simulink model "robotLQG_sim"  (R2026b)
settings: Solver=ode45  StopTime=Tstop  MaxStep=0.002  RelTol=1e-6
PreLoadFcn:
  | robotLQG_setup_AIgen;
InitFcn:
  | robotLQG_setup_AIgen;
values from neighbouring files (symbols this model uses):
  alphaMax = lim.alphaMax    [robotLQG_setup_AIgen.m]    (also in stepperLimits_AIgen.m = alphaBox(k))
  gyroNoiseVar = sensorNonIdeal*sigGyro^2    (= 1.21846967915e-05)    [robotLQG_setup_AIgen.m]
  K = lqrd(Ai, Bi, Q, R, Ts)    [robotLQG_setup_AIgen.m]    (also in robotPoleExplorer_AIgen.m = lqr(me.A, me.B, Q, Rw); solveDARE_AIgen.m = (R + B'*P*B) \ (B'*P*A + N'))
  kest = kalmd(ss(A1,[B1, B1],C1,zeros(2,2)),1/24,((pi/180)^2)*[1/24 0; 0 5E-6],Ts)    [controller_lqg_ia.m]    (also in discreteKalman_AIgen.m = struct('A', Ad - L*C, 'B', [Bd - L*D, L], 'L', L,           ; robotLQG_setup_AIgen.m = kalmd(ss(A, [B, G], C, [D, zeros(3, 2)]), Qn, Rn, Ts))
  omegaMax = lim.omegaMax    [robotLQG_setup_AIgen.m]    (also in stepperLimits_AIgen.m = w(k))
  p = struct('mc', mc, 'Jc', Jc, 'mw', mw, 'Jw', Jw, 'l', l, 'r', r,                         'g', 9.81,                         'Jr', 2*Jrotor,                         'b_phi', 0,                         'b_theta', 0)    [classBalancingRobotFlowLinear_AIgen.m]    (also in classBalancingRobotRigLinear_AIgen.m = classBalancingRobotFlowLinear_AIgen.estimatedParameters(); fitRigFall_AIgen.m = c(nRun + 1:end); robotLQG_setup_AIgen.m = [robot.mc; robot.Jc; robot.mw; robot.Jw; robot.l; robot.r; r)
  phiRefRate = 2    [robotLQG_setup_AIgen.m]
  phiRefStepTime = 3    [robotLQG_setup_AIgen.m]
  thetaBiasUsed = sensorNonIdeal*thetaBias    (= 0.0261799387799)    [robotLQG_setup_AIgen.m]
  thetaNoiseVar = sensorNonIdeal*sigTheta^2    (= 1.21846967915e-05)    [robotLQG_setup_AIgen.m]
  Ts = 0.002    [robotLQG_setup_AIgen.m]
  x0 = [0; theta0; obj.momentum(0, dtheta0)]    [classBalancingRobotRigLinear_AIgen.m]    (also in robotLQG_setup_AIgen.m = [0; 5*pi/180; 0])
  xhat0 = [0; x0(2) + thetaBiasUsed; 0]    [robotLQG_setup_AIgen.m]
  zLimit = 0.5*alphaMax/abs(Kz)    [robotLQG_setup_AIgen.m]
undefined symbols (not defined in the file or in its folder): DiscIntNeverNeededParam
settings Model: Creator=61404  LastModifiedBy=61404

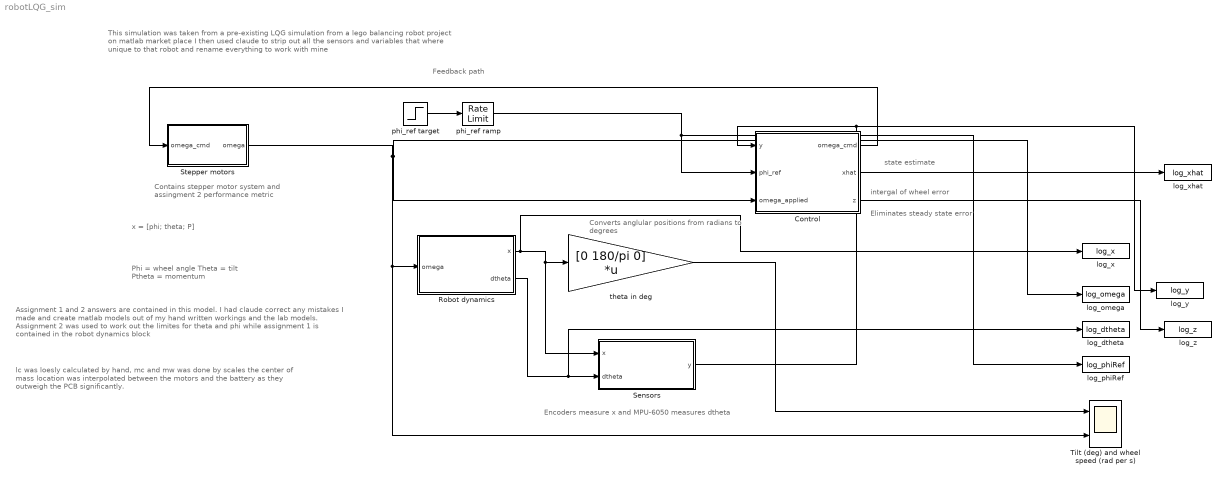
== system robotLQG_sim ==
  note: lc was loesly calculated by hand, mc and mw was done by scales
      | the center of mass location was interpolated between the motors and the
      | battery as they outweigh the PCB significantly.
  note: Assignment 1 and 2 answers are contained in this model.
      | I had claude correct any mistakes I made and create matlab models out of my
      | hand written workings and the lab models. Assignment 2 was used to work out
      | the limites for theta and phi while assignment 1 is contained in the robot dynamics block
  note: Eliminates steady state error
  note: intergal of wheel error
  note: state estimate
  note: Phi = wheel angle
      | Theta = tilt
      | Ptheta = momentum
  note: x = [phi;
      | 	theta;
      | 	P]
  note: This simulation was taken from a pre-existing LQG simulation from a lego balancing robot project on matlab market place
      | I then used claude to strip out all the sensors and variables that where unique to that robot and rename everything to work with mine
  note: Encoders measure x and MPU-6050 measures dtheta
  note: Feedback path
  note: Converts anglular positions from radians to
      | degrees
  note: Contains stepper motor system
      | and assingment 2 performance metric
  Control : Subsystem
  Robot dynamics : Subsystem
  Sensors : Subsystem
  Stepper motors : Subsystem
  Tilt (deg) and wheel speed (rad per s) : Scope  NumInputPorts=2
  log_dtheta : ToWorkspace  VariableName=log_dtheta  SaveFormat=Structure With Time  SampleTime=Ts
  log_omega : ToWorkspace  VariableName=log_omega  SaveFormat=Structure With Time  SampleTime=Ts
  log_phiRef : ToWorkspace  VariableName=log_phiRef  SaveFormat=Structure With Time  SampleTime=Ts
  log_x : ToWorkspace  VariableName=log_x  SaveFormat=Structure With Time  SampleTime=Ts
  log_xhat : ToWorkspace  VariableName=log_xhat  SaveFormat=Structure With Time  SampleTime=Ts
  log_y : ToWorkspace  VariableName=log_y  SaveFormat=Structure With Time  SampleTime=Ts
  log_z : ToWorkspace  VariableName=log_z  SaveFormat=Structure With Time  SampleTime=Ts
  phi_ref ramp : RateLimiter  RisingSlewLimit=phiRefRate  FallingSlewLimit=-phiRefRate  SampleTimeMode=inherited
  phi_ref target : Step  Time=phiRefStepTime  FinalValue=phiRefStep  SampleTime=Ts
  theta in deg : Gain  Gain=[0 180/pi 0]  Multiplication=Matrix(K*u)
  wires:
  Robot dynamics/1(x) -> Sensors/1(x), theta in deg/1, log_x/1
  Stepper motors/1(omega) -> Tilt (deg) and wheel speed (rad per s)/2, Robot dynamics/1(omega), Control/3(omega_applied), log_omega/1
  phi_ref target/1 -> phi_ref ramp/1
  Sensors/1(y) -> Control/1(y), log_y/1
  Control/1(omega_cmd) -> Stepper motors/1(omega_cmd)
  Robot dynamics/2(dtheta) -> Sensors/2(dtheta), log_dtheta/1
  phi_ref ramp/1 -> Control/2(phi_ref), log_phiRef/1
  theta in deg/1 -> Tilt (deg) and wheel speed (rad per s)/1
  Control/2(xhat) -> log_xhat/1
  Control/3(z) -> log_z/1

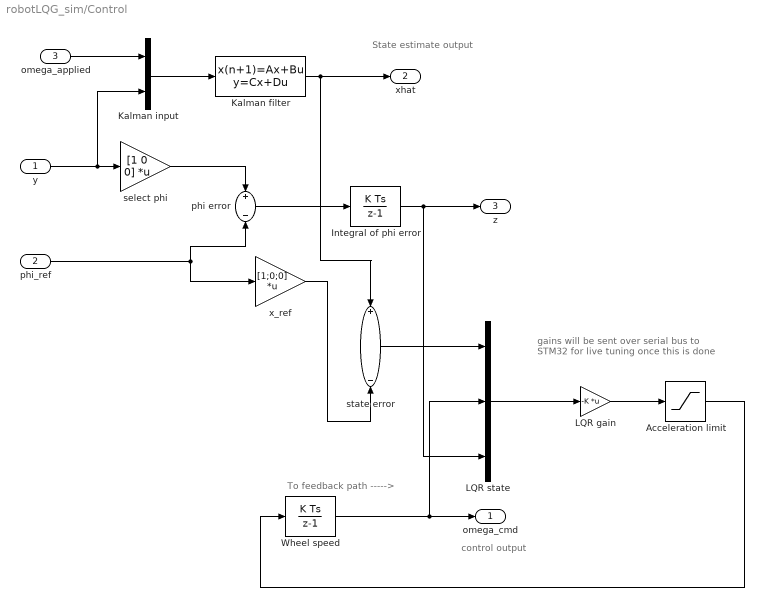
== system robotLQG_sim/Control ==
  note: State estimate output
  note: control output
  note: To feedback path ----->
  note: gains will be sent over serial bus to
      | STM32 for live tuning once this is done
  y : Inport
  phi_ref : Inport  Port=2
  omega_applied : Inport  Port=3
  Acceleration limit : Saturate  UpperLimit=alphaMax  LowerLimit=-alphaMax
  Integral of phi error : DiscreteIntegrator  SampleTime=Ts  LimitOutput=on  UpperSaturationLimit=zLimit  LowerSaturationLimit=-zLimit  ICPrevOutput=DiscIntNeverNeededParam  ICPrevScaledInput=DiscIntNeverNeededParam
  Kalman filter : DiscreteStateSpace  A=kest.A  B=kest.B  C=eye(3)  D=zeros(3,4)  InitialCondition=xhat0  SampleTime=Ts
  Kalman input : Mux  Inputs=2
  LQR gain : Gain  Gain=-K  Multiplication=Matrix(K*u)
  LQR state : Mux  Inputs=3
  Wheel speed : DiscreteIntegrator  SampleTime=Ts  LimitOutput=on  UpperSaturationLimit=omegaMax  LowerSaturationLimit=-omegaMax  ICPrevOutput=DiscIntNeverNeededParam  ICPrevScaledInput=DiscIntNeverNeededParam
  phi error : Sum  Inputs=+-
  select phi : Gain  Gain=[1 0 0]  Multiplication=Matrix(K*u)
  state error : Sum  Inputs=+-
  x_ref : Gain  Gain=[1;0;0]  Multiplication=Matrix(K*u)
  omega_cmd : Outport
  xhat : Outport  Port=2
  z : Outport  Port=3
  wires:
  phi_ref/1 -> phi error/2, x_ref/1
  y/1 -> Kalman input/2, select phi/1
  omega_applied/1 -> Kalman input/1
  Kalman input/1 -> Kalman filter/1
  select phi/1 -> phi error/1
  phi error/1 -> Integral of phi error/1
  x_ref/1 -> state error/2
  Kalman filter/1 -> state error/1, xhat/1
  LQR gain/1 -> Acceleration limit/1
  LQR state/1 -> LQR gain/1
  Integral of phi error/1 -> LQR state/3, z/1
  state error/1 -> LQR state/1
  Wheel speed/1 -> LQR state/2, omega_cmd/1
  Acceleration limit/1 -> Wheel speed/1

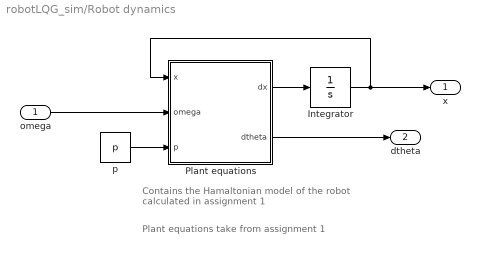
== system robotLQG_sim/Robot dynamics ==
  note: Plant equations take from assignment 1
  note: Contains the Hamaltonian model of the robot
      | calculated in assignment 1
  omega : Inport
  Integrator : Integrator  InitialCondition=x0
  Plant equations : MATLAB Function  TreatAsAtomicUnit=on
  p : Constant  Value=p
  x : Outport
  dtheta : Outport  Port=2
  wires:
  p/1 -> Plant equations/3(p)
  omega/1 -> Plant equations/2(omega)
  Plant equations/1(dx) -> Integrator/1
  Plant equations/2(dtheta) -> dtheta/1
  Integrator/1 -> Plant equations/1(x), x/1

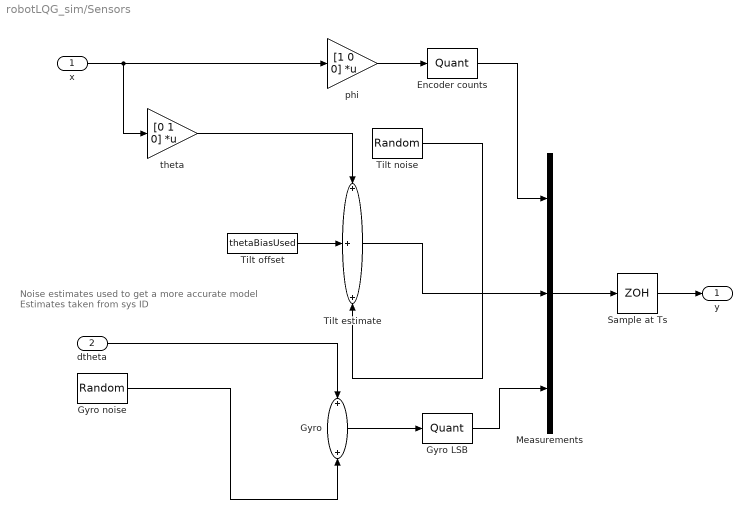
== system robotLQG_sim/Sensors ==
  note: Noise estimates used to get a more accurate model
      | Estimates taken from sys ID
  x : Inport
  dtheta : Inport  Port=2
  Encoder counts : Quantizer  QuantizationInterval=encQ
  Gyro : Sum
  Gyro LSB : Quantizer  QuantizationInterval=gyroQ
  Gyro noise : RandomNumber  Variance=gyroNoiseVar  Seed=2  SampleTime=Ts
  Measurements : Mux  Inputs=3
  Sample at Ts : ZeroOrderHold  SampleTime=Ts
  Tilt estimate : Sum  Inputs=+++
  Tilt noise : RandomNumber  Variance=thetaNoiseVar  Seed=1  SampleTime=Ts
  Tilt offset : Constant  Value=thetaBiasUsed
  phi : Gain  Gain=[1 0 0]  Multiplication=Matrix(K*u)
  theta : Gain  Gain=[0 1 0]  Multiplication=Matrix(K*u)
  y : Outport
  wires:
  phi/1 -> Encoder counts/1
  dtheta/1 -> Gyro/1
  x/1 -> phi/1, theta/1
  Gyro/1 -> Gyro LSB/1
  Tilt estimate/1 -> Measurements/2
  Tilt offset/1 -> Tilt estimate/2
  Measurements/1 -> Sample at Ts/1
  theta/1 -> Tilt estimate/1
  Tilt noise/1 -> Tilt estimate/3
  Encoder counts/1 -> Measurements/1
  Gyro noise/1 -> Gyro/2
  Gyro LSB/1 -> Measurements/3
  Sample at Ts/1 -> y/1

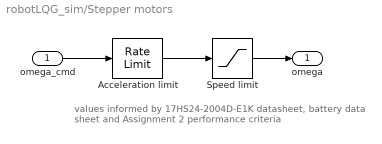
== system robotLQG_sim/Stepper motors ==
  note: values informed by 17HS24-2004D-E1K
      | datasheet, battery data sheet and Assignment 2 performance
      | criteria
  omega_cmd : Inport
  Acceleration limit : RateLimiter  RisingSlewLimit=alphaMax  FallingSlewLimit=-alphaMax  SampleTimeMode=inherited
  Speed limit : Saturate  UpperLimit=omegaMax  LowerLimit=-omegaMax
  omega : Outport
  wires:
  omega_cmd/1 -> Acceleration limit/1
  Speed limit/1 -> omega/1
  Acceleration limit/1 -> Speed limit/1

== matlab function robotLQG_sim/Robot dynamics/Plant equations ==
  data: x input; dx output; omega input; p input; dtheta output
function [dx, dtheta] = plant(x, omega, p)
% Flow-source model of the robot: robotFlowPlant_AIgen.m (AI-generated, Claude).
% x = [phi; theta; ptheta], omega = stepper speed relative to the chassis.
[dx, dtheta] = robotFlowPlant_AIgen(x, omega, p);
